simulink model "fft_biplex_real_4x_delay_bram_test"  (Simulink 7.4)
settings: Solver=VariableStepDiscrete  StartTime=0.0  StopTime=256  RelTol=1e-3
libraries: xbsIndex_r4 x596, casper_library_misc x36, casper_library_delays x8, casper_library_ffts_twiddle x1, simulink x1
(part 3 of 6)

== system fft_biplex_real_4x_delay_bram_test/fft_biplex_real_4x/biplex_core/fft_stage_3 ==
  in1 : Inport  OutDataType=sfix(16)  OutScaling=2^0
  in2 : Inport  Port=2  OutDataType=sfix(16)  OutScaling=2^0
  of_in : Inport  Port=3  OutDataType=sfix(16)  OutScaling=2^0
  sync : Inport  Port=4  OutDataType=sfix(16)  OutScaling=2^0
  shift : Inport  Port=5  OutDataType=sfix(16)  OutScaling=2^0
  Counter : xbsIndex_r4/Counter  cnt_type=Free Running  cnt_to=Inf  operation=Up  start_count=0  cnt_by_val=1  arith_type=Unsigned  n_bits=FFTSize-FFTStage+1  bin_pt=0  load_pin=off  rst=on  en=off  explicit_period=off  period=1  dbl_ovrd=off  use_behavioral_HDL=off  implementation=Fabric  use_rpm=off  block_type=counter
      settings: xl_area=[0, 0, 0, 0, 0, 0, 0]  block_version=9.1.01
  Delay : xbsIndex_r4/Delay  en=off  latency=1  dbl_ovrd=off  reg_retiming=off  block_type=delay
      settings: xl_area=[0, 0, 0, 0, 0, 0, 0]  block_version=9.1.01
  Logical1 : xbsIndex_r4/Logical  logical_function=OR  inputs=2  en=off  latency=1  precision=Full  arith_type=Unsigned  n_bits=8  bin_pt=2  align_bp=on  dbl_ovrd=off  block_type=logical
      settings: xl_area=[0, 0, 0, 0, 0, 0, 0]  block_version=9.1.01
  Mux : xbsIndex_r4/Mux  inputs=2  en=off  latency=1  precision=Full  arith_type="Signed  (2's comp)"  n_bits=8  bin_pt=2  quantization=Truncate  overflow=Wrap  dbl_ovrd=off  block_type=mux
      settings: xl_area=[0, 0, 0, 0, 0, 0, 0]  block_version=9.1.01
  Mux1 : xbsIndex_r4/Mux  inputs=2  en=off  latency=1  precision=Full  arith_type="Signed  (2's comp)"  n_bits=8  bin_pt=2  quantization=Truncate  overflow=Wrap  dbl_ovrd=off  block_type=mux
      settings: xl_area=[0, 0, 0, 0, 0, 0, 0]  block_version=9.1.01
  Slice : xbsIndex_r4/Slice  nbits=1  boolean_output=on  mode=Lower Bit Location + Width  bit1=-(FFTStage - 1)  base1=MSB of Input  bit0=FFTStage - 1  base0=LSB of Input  dbl_ovrd=off  block_type=slice
      settings: infoedit="Extracts a given range of bits from each input sample and presents it at the output.  The output type is ordinarily unsigned with binary point at zero, but can be Boolean when the slice is one bit wide.<P><P>Hardware notes: In hardware this block costs nothing."  block_version=9.1.01
  Slice1 : xbsIndex_r4/Slice  nbits=1  boolean_output=off  mode=Upper Bit Location + Width  bit1=0  base1=MSB of Input  bit0=0  base0=LSB of Input  dbl_ovrd=off  block_type=slice
      settings: infoedit="Extracts a given range of bits from each input sample and presents it at the output.  The output type is ordinarily unsigned with binary point at zero, but can be Boolean when the slice is one bit wide.<P><P>Hardware notes: In hardware this block costs nothing."  block_version=9.1.01
  butterfly_direct : Subsystem  AncestorBlock=casper_library_ffts/butterfly_direct  mask(butterfly_direct){biplex=on, FFTSize=5, Coeffs=getfield( getfield( get_param( gcb,'UserData' ), 'parameters'),'Coeffs'), StepPeriod=2, coeff_bit_width=16, input_bit_width=16, downshift=off, add_latency=1, mult_latency=3, bram_latency=1, conv_latency=2, quantization=Truncate, overflow=Saturate, arch=Virtex2Pro, opt_target=multipliers, coeffs_bram=off, use_hdl=on, use_embedded=off, hardcode_shifts=off, dsp48_adders=off}
      mask prompts: biplex "Used in biplex FFT"; FFTSize "Size of FFT: (2^? pts)"; Coeffs "Coefficients: (0 to 2^(FFTSize-1)-1)"; StepPeriod "Coefficient Step Period: (2^?)"; coeff_bit_width "Coefficient Bit Width"; input_bit_width "Input/Output Bit Width:"; add_latency "Add Latency"; mult_latency "Mult Latency"; bram_latency "BRAM Latency"; conv_latency "Convert latency"; quantization "Quantization Behavior"; overflow "Overflow Behavior"; arch "Architecture"; opt_target "Use less"; coeffs_bram "Store coefficients in BRAM"; use_hdl "Use behavioural HDL for multipliers"; use_embedded "Use embedded multipliers"; hardcode_shifts "Hardcode shift schedule"; dsp48_adders "Use DSP48s for adders"
      mask help: FFT internal block.
      mask init: same as fft_biplex_real_4x_delay_bram_test/fft_biplex_real_4x/biplex_core/fft_stage_1/butterfly_direct
      settings: AttributesFormatString=|
      | twiddle_general_3mult
      | coeffs in slices
      mask StyleString: checkbox,edit,edit,edit,edit,edit,checkbox,edit,edit,edit,edit,popup(Truncate|Round  (unbiased: +/- Inf)|Round  (unbiased: Even Values)),popup(Wrap|Saturate|Error),popup(Virtex2Pro|Virtex5),popup(logic|multipliers),checkbox,checkbox,checkbox,checkbox,checkbox
      mask CallbackString:
      | ||Coeffs = get_param(gcb, 'Coeffs');
      | if (length(eval(Coeffs)) == 1),
      |     set_param_state(gcb, 'StepPeriod', 'off');
      |     set_param_state(gcb, 'coeffs_bram', 'off');
      |     set_param_state(gcb, 'coeff_bit_width', 'off');
      | else
      |     set_param_state(gcb, 'StepPeriod', 'on');
      |     set_param_state(gcb, 'coeffs_bram', 'on');
      |     set_param_state(gcb, 'coeff_bit_width', 'on');
      | end|||||||||||fft_callback_arch(gcb);|||% make mutually exclusive with use_embedded.
      | 
      | use_hdl = get_param(gcb, 'use_hdl');
      | if strcmp(use_hdl, 'on'),
      |     set_param_state(gcb, 'use_embedded', 'off');
      | else
      |     set_param_state(gcb, 'use_embedded', 'on');
      | end|% make mutually exclusive with use_hdl.
      | 
      | use_hdl = get_param(gcb, 'use_embedded');
      | if strcmp(use_hdl, 'on'),
      |     set_param_state(gcb, 'use_hdl', 'off');
      | else
      |     set_param_state(gcb, 'use_hdl', 'on');
      | end|hardcode_shifts = get_param(gcb, 'hardcode_shifts');
      | set_param_state(gcb, 'downshift', hardcode_shifts);|fft_callback_dsp48_adders(gcb);
      mask TabNameString: Basic,Basic,Basic,Basic,Basic,Basic,Basic,Latency,Latency,Latency,Latency,Implementation,Implementation,Implementation,Implementation,Implementation,Implementation,Implementation,Implementation,Implementation
  delay_b : Subsystem  AncestorBlock=casper_library_delays/delay_slr  mask(delay_slr){DelayLen=2^(FFTSize-FFTStage)}
      mask prompts: DelayLen "Delay by:"
      mask help: A delay block that uses slices (SLR16s) for its storage.
      mask Help: eval('xlWeb(''http://casper.berkeley.edu/wiki/Delay_slr'')')
  delay_f : Subsystem  AncestorBlock=casper_library_delays/delay_slr  mask(delay_slr){DelayLen=2^(FFTSize-FFTStage)}
      mask prompts: DelayLen "Delay by:"
      mask help: A delay block that uses slices (SLR16s) for its storage.
      mask Help: eval('xlWeb(''http://casper.berkeley.edu/wiki/Delay_slr'')')
  sync_delay : casper_library_delays/sync_delay  SystemSampleTime=-1  DelayLen=2^(FFTSize - FFTStage)
  out1 : Outport  OutDataType=sfix(16)  OutScaling=2^0
  out2 : Outport  Port=2  OutDataType=sfix(16)  OutScaling=2^0
  of : Outport  Port=3  OutDataType=sfix(16)  OutScaling=2^0
  sync_out : Outport  Port=4  OutDataType=sfix(16)  OutScaling=2^0
  wires:
  shift/1 -> Slice/1
  of_in/1 -> Logical1/2
  Logical1/1 -> of/1
  Delay/1 -> sync_delay/1
  sync/1 -> Counter/1, Delay/1
  Counter/1 -> Slice1/1
  Mux/1 -> butterfly_direct/2(b)
  Mux1/1 -> delay_b/1(In1)
  delay_f/1(Out1) -> Mux1/3, Mux/2
  in1/1 -> Mux/3, Mux1/2
  Slice1/1 -> Mux/1, Mux1/1
  in2/1 -> delay_f/1(In1)
  delay_b/1(Out1) -> butterfly_direct/1(a)
  sync_delay/1 -> butterfly_direct/3(sync)
  Slice/1 -> butterfly_direct/4(shift)
  butterfly_direct/1(a+bw) -> out1/1
  butterfly_direct/2(a-bw) -> out2/1
  butterfly_direct/3(of) -> Logical1/1
  butterfly_direct/4(sync_out) -> sync_out/1

== system fft_biplex_real_4x_delay_bram_test/fft_biplex_real_4x/biplex_core/fft_stage_4 ==
  in1 : Inport  OutDataType=sfix(16)  OutScaling=2^0
  in2 : Inport  Port=2  OutDataType=sfix(16)  OutScaling=2^0
  of_in : Inport  Port=3  OutDataType=sfix(16)  OutScaling=2^0
  sync : Inport  Port=4  OutDataType=sfix(16)  OutScaling=2^0
  shift : Inport  Port=5  OutDataType=sfix(16)  OutScaling=2^0
  Counter : xbsIndex_r4/Counter  cnt_type=Free Running  cnt_to=Inf  operation=Up  start_count=0  cnt_by_val=1  arith_type=Unsigned  n_bits=FFTSize-FFTStage+1  bin_pt=0  load_pin=off  rst=on  en=off  explicit_period=off  period=1  dbl_ovrd=off  use_behavioral_HDL=off  implementation=Fabric  use_rpm=off  block_type=counter
      settings: xl_area=[0, 0, 0, 0, 0, 0, 0]  block_version=9.1.01
  Delay : xbsIndex_r4/Delay  en=off  latency=1  dbl_ovrd=off  reg_retiming=off  block_type=delay
      settings: xl_area=[0, 0, 0, 0, 0, 0, 0]  block_version=9.1.01
  Logical1 : xbsIndex_r4/Logical  logical_function=OR  inputs=2  en=off  latency=1  precision=Full  arith_type=Unsigned  n_bits=8  bin_pt=2  align_bp=on  dbl_ovrd=off  block_type=logical
      settings: xl_area=[0, 0, 0, 0, 0, 0, 0]  block_version=9.1.01
  Mux : xbsIndex_r4/Mux  inputs=2  en=off  latency=1  precision=Full  arith_type="Signed  (2's comp)"  n_bits=8  bin_pt=2  quantization=Truncate  overflow=Wrap  dbl_ovrd=off  block_type=mux
      settings: xl_area=[0, 0, 0, 0, 0, 0, 0]  block_version=9.1.01
  Mux1 : xbsIndex_r4/Mux  inputs=2  en=off  latency=1  precision=Full  arith_type="Signed  (2's comp)"  n_bits=8  bin_pt=2  quantization=Truncate  overflow=Wrap  dbl_ovrd=off  block_type=mux
      settings: xl_area=[0, 0, 0, 0, 0, 0, 0]  block_version=9.1.01
  Slice : xbsIndex_r4/Slice  nbits=1  boolean_output=on  mode=Lower Bit Location + Width  bit1=-(FFTStage - 1)  base1=MSB of Input  bit0=FFTStage - 1  base0=LSB of Input  dbl_ovrd=off  block_type=slice
      settings: infoedit="Extracts a given range of bits from each input sample and presents it at the output.  The output type is ordinarily unsigned with binary point at zero, but can be Boolean when the slice is one bit wide.<P><P>Hardware notes: In hardware this block costs nothing."  block_version=9.1.01
  Slice1 : xbsIndex_r4/Slice  nbits=1  boolean_output=off  mode=Upper Bit Location + Width  bit1=0  base1=MSB of Input  bit0=0  base0=LSB of Input  dbl_ovrd=off  block_type=slice
      settings: infoedit="Extracts a given range of bits from each input sample and presents it at the output.  The output type is ordinarily unsigned with binary point at zero, but can be Boolean when the slice is one bit wide.<P><P>Hardware notes: In hardware this block costs nothing."  block_version=9.1.01
  butterfly_direct : Subsystem  AncestorBlock=casper_library_ffts/butterfly_direct  mask(butterfly_direct){biplex=on, FFTSize=5, Coeffs=getfield( getfield( get_param( gcb,'UserData' ), 'parameters'),'Coeffs'), StepPeriod=1, coeff_bit_width=16, input_bit_width=16, downshift=off, add_latency=1, mult_latency=3, bram_latency=1, conv_latency=2, quantization=Truncate, overflow=Saturate, arch=Virtex2Pro, opt_target=multipliers, coeffs_bram=off, use_hdl=on, use_embedded=off, hardcode_shifts=off, dsp48_adders=off}
      mask prompts: biplex "Used in biplex FFT"; FFTSize "Size of FFT: (2^? pts)"; Coeffs "Coefficients: (0 to 2^(FFTSize-1)-1)"; StepPeriod "Coefficient Step Period: (2^?)"; coeff_bit_width "Coefficient Bit Width"; input_bit_width "Input/Output Bit Width:"; add_latency "Add Latency"; mult_latency "Mult Latency"; bram_latency "BRAM Latency"; conv_latency "Convert latency"; quantization "Quantization Behavior"; overflow "Overflow Behavior"; arch "Architecture"; opt_target "Use less"; coeffs_bram "Store coefficients in BRAM"; use_hdl "Use behavioural HDL for multipliers"; use_embedded "Use embedded multipliers"; hardcode_shifts "Hardcode shift schedule"; dsp48_adders "Use DSP48s for adders"
      mask help: FFT internal block.
      mask init: same as fft_biplex_real_4x_delay_bram_test/fft_biplex_real_4x/biplex_core/fft_stage_1/butterfly_direct
      settings: AttributesFormatString=|
      | twiddle_general_3mult
      | coeffs in slices
      mask StyleString: checkbox,edit,edit,edit,edit,edit,checkbox,edit,edit,edit,edit,popup(Truncate|Round  (unbiased: +/- Inf)|Round  (unbiased: Even Values)),popup(Wrap|Saturate|Error),popup(Virtex2Pro|Virtex5),popup(logic|multipliers),checkbox,checkbox,checkbox,checkbox,checkbox
      mask CallbackString:
      | ||Coeffs = get_param(gcb, 'Coeffs');
      | if (length(eval(Coeffs)) == 1),
      |     set_param_state(gcb, 'StepPeriod', 'off');
      |     set_param_state(gcb, 'coeffs_bram', 'off');
      |     set_param_state(gcb, 'coeff_bit_width', 'off');
      | else
      |     set_param_state(gcb, 'StepPeriod', 'on');
      |     set_param_state(gcb, 'coeffs_bram', 'on');
      |     set_param_state(gcb, 'coeff_bit_width', 'on');
      | end|||||||||||fft_callback_arch(gcb);|||% make mutually exclusive with use_embedded.
      | 
      | use_hdl = get_param(gcb, 'use_hdl');
      | if strcmp(use_hdl, 'on'),
      |     set_param_state(gcb, 'use_embedded', 'off');
      | else
      |     set_param_state(gcb, 'use_embedded', 'on');
      | end|% make mutually exclusive with use_hdl.
      | 
      | use_hdl = get_param(gcb, 'use_embedded');
      | if strcmp(use_hdl, 'on'),
      |     set_param_state(gcb, 'use_hdl', 'off');
      | else
      |     set_param_state(gcb, 'use_hdl', 'on');
      | end|hardcode_shifts = get_param(gcb, 'hardcode_shifts');
      | set_param_state(gcb, 'downshift', hardcode_shifts);|fft_callback_dsp48_adders(gcb);
      mask TabNameString: Basic,Basic,Basic,Basic,Basic,Basic,Basic,Latency,Latency,Latency,Latency,Implementation,Implementation,Implementation,Implementation,Implementation,Implementation,Implementation,Implementation,Implementation
  delay_b : Subsystem  AncestorBlock=casper_library_delays/delay_slr  mask(delay_slr){DelayLen=2^(FFTSize-FFTStage)}
      mask prompts: DelayLen "Delay by:"
      mask help: A delay block that uses slices (SLR16s) for its storage.
      mask Help: eval('xlWeb(''http://casper.berkeley.edu/wiki/Delay_slr'')')
  delay_f : Subsystem  AncestorBlock=casper_library_delays/delay_slr  mask(delay_slr){DelayLen=2^(FFTSize-FFTStage)}
      mask prompts: DelayLen "Delay by:"
      mask help: A delay block that uses slices (SLR16s) for its storage.
      mask Help: eval('xlWeb(''http://casper.berkeley.edu/wiki/Delay_slr'')')
  sync_delay : casper_library_delays/sync_delay  SystemSampleTime=-1  DelayLen=2^(FFTSize - FFTStage)
  out1 : Outport  OutDataType=sfix(16)  OutScaling=2^0
  out2 : Outport  Port=2  OutDataType=sfix(16)  OutScaling=2^0
  of : Outport  Port=3  OutDataType=sfix(16)  OutScaling=2^0
  sync_out : Outport  Port=4  OutDataType=sfix(16)  OutScaling=2^0
  wires:
  shift/1 -> Slice/1
  of_in/1 -> Logical1/2
  Logical1/1 -> of/1
  Delay/1 -> sync_delay/1
  sync/1 -> Counter/1, Delay/1
  Counter/1 -> Slice1/1
  Mux/1 -> butterfly_direct/2(b)
  Mux1/1 -> delay_b/1(In1)
  delay_f/1(Out1) -> Mux1/3, Mux/2
  in1/1 -> Mux/3, Mux1/2
  Slice1/1 -> Mux/1, Mux1/1
  in2/1 -> delay_f/1(In1)
  delay_b/1(Out1) -> butterfly_direct/1(a)
  sync_delay/1 -> butterfly_direct/3(sync)
  Slice/1 -> butterfly_direct/4(shift)
  butterfly_direct/1(a+bw) -> out1/1
  butterfly_direct/2(a-bw) -> out2/1
  butterfly_direct/3(of) -> Logical1/1
  butterfly_direct/4(sync_out) -> sync_out/1

== system fft_biplex_real_4x_delay_bram_test/fft_biplex_real_4x/biplex_core/fft_stage_5 ==
  in1 : Inport  OutDataType=sfix(16)  OutScaling=2^0
  in2 : Inport  Port=2  OutDataType=sfix(16)  OutScaling=2^0
  of_in : Inport  Port=3  OutDataType=sfix(16)  OutScaling=2^0
  sync : Inport  Port=4  OutDataType=sfix(16)  OutScaling=2^0
  shift : Inport  Port=5  OutDataType=sfix(16)  OutScaling=2^0
  Counter : xbsIndex_r4/Counter  cnt_type=Free Running  cnt_to=Inf  operation=Up  start_count=0  cnt_by_val=1  arith_type=Unsigned  n_bits=FFTSize-FFTStage+1  bin_pt=0  load_pin=off  rst=on  en=off  explicit_period=off  period=1  dbl_ovrd=off  use_behavioral_HDL=off  implementation=Fabric  use_rpm=off  block_type=counter
      settings: xl_area=[0, 0, 0, 0, 0, 0, 0]  block_version=9.1.01
  Delay : xbsIndex_r4/Delay  en=off  latency=1  dbl_ovrd=off  reg_retiming=off  block_type=delay
      settings: xl_area=[0, 0, 0, 0, 0, 0, 0]  block_version=9.1.01
  Logical1 : xbsIndex_r4/Logical  logical_function=OR  inputs=2  en=off  latency=1  precision=Full  arith_type=Unsigned  n_bits=8  bin_pt=2  align_bp=on  dbl_ovrd=off  block_type=logical
      settings: xl_area=[0, 0, 0, 0, 0, 0, 0]  block_version=9.1.01
  Mux : xbsIndex_r4/Mux  inputs=2  en=off  latency=1  precision=Full  arith_type="Signed  (2's comp)"  n_bits=8  bin_pt=2  quantization=Truncate  overflow=Wrap  dbl_ovrd=off  block_type=mux
      settings: xl_area=[0, 0, 0, 0, 0, 0, 0]  block_version=9.1.01
  Mux1 : xbsIndex_r4/Mux  inputs=2  en=off  latency=1  precision=Full  arith_type="Signed  (2's comp)"  n_bits=8  bin_pt=2  quantization=Truncate  overflow=Wrap  dbl_ovrd=off  block_type=mux
      settings: xl_area=[0, 0, 0, 0, 0, 0, 0]  block_version=9.1.01
  Slice : xbsIndex_r4/Slice  nbits=1  boolean_output=on  mode=Lower Bit Location + Width  bit1=-(FFTStage - 1)  base1=MSB of Input  bit0=FFTStage - 1  base0=LSB of Input  dbl_ovrd=off  block_type=slice
      settings: infoedit="Extracts a given range of bits from each input sample and presents it at the output.  The output type is ordinarily unsigned with binary point at zero, but can be Boolean when the slice is one bit wide.<P><P>Hardware notes: In hardware this block costs nothing."  block_version=9.1.01
  Slice1 : xbsIndex_r4/Slice  nbits=1  boolean_output=off  mode=Upper Bit Location + Width  bit1=0  base1=MSB of Input  bit0=0  base0=LSB of Input  dbl_ovrd=off  block_type=slice
      settings: infoedit="Extracts a given range of bits from each input sample and presents it at the output.  The output type is ordinarily unsigned with binary point at zero, but can be Boolean when the slice is one bit wide.<P><P>Hardware notes: In hardware this block costs nothing."  block_version=9.1.01
  butterfly_direct : Subsystem  AncestorBlock=casper_library_ffts/butterfly_direct  mask(butterfly_direct){biplex=on, FFTSize=5, Coeffs=getfield( getfield( get_param( gcb,'UserData' ), 'parameters'),'Coeffs'), StepPeriod=0, coeff_bit_width=16, input_bit_width=16, downshift=off, add_latency=1, mult_latency=3, bram_latency=1, conv_latency=2, quantization=Truncate, overflow=Saturate, arch=Virtex2Pro, opt_target=multipliers, coeffs_bram=off, use_hdl=off, use_embedded=on, hardcode_shifts=off, dsp48_adders=off}
      mask prompts: biplex "Used in biplex FFT"; FFTSize "Size of FFT: (2^? pts)"; Coeffs "Coefficients: (0 to 2^(FFTSize-1)-1)"; StepPeriod "Coefficient Step Period: (2^?)"; coeff_bit_width "Coefficient Bit Width"; input_bit_width "Input/Output Bit Width:"; add_latency "Add Latency"; mult_latency "Mult Latency"; bram_latency "BRAM Latency"; conv_latency "Convert latency"; quantization "Quantization Behavior"; overflow "Overflow Behavior"; arch "Architecture"; opt_target "Use less"; coeffs_bram "Store coefficients in BRAM"; use_hdl "Use behavioural HDL for multipliers"; use_embedded "Use embedded multipliers"; hardcode_shifts "Hardcode shift schedule"; dsp48_adders "Use DSP48s for adders"
      mask help: FFT internal block.
      mask init: same as fft_biplex_real_4x_delay_bram_test/fft_biplex_real_4x/biplex_core/fft_stage_1/butterfly_direct
      settings: AttributesFormatString=|
      | twiddle_general_3mult
      | coeffs in slices
      mask StyleString: checkbox,edit,edit,edit,edit,edit,checkbox,edit,edit,edit,edit,popup(Truncate|Round  (unbiased: +/- Inf)|Round  (unbiased: Even Values)),popup(Wrap|Saturate|Error),popup(Virtex2Pro|Virtex5),popup(logic|multipliers),checkbox,checkbox,checkbox,checkbox,checkbox
      mask CallbackString:
      | ||Coeffs = get_param(gcb, 'Coeffs');
      | if (length(eval(Coeffs)) == 1),
      |     set_param_state(gcb, 'StepPeriod', 'off');
      |     set_param_state(gcb, 'coeffs_bram', 'off');
      |     set_param_state(gcb, 'coeff_bit_width', 'off');
      | else
      |     set_param_state(gcb, 'StepPeriod', 'on');
      |     set_param_state(gcb, 'coeffs_bram', 'on');
      |     set_param_state(gcb, 'coeff_bit_width', 'on');
      | end|||||||||||fft_callback_arch(gcb);|||% make mutually exclusive with use_embedded.
      | 
      | use_hdl = get_param(gcb, 'use_hdl');
      | if strcmp(use_hdl, 'on'),
      |     set_param_state(gcb, 'use_embedded', 'off');
      | else
      |     set_param_state(gcb, 'use_embedded', 'on');
      | end|% make mutually exclusive with use_hdl.
      | 
      | use_hdl = get_param(gcb, 'use_embedded');
      | if strcmp(use_hdl, 'on'),
      |     set_param_state(gcb, 'use_hdl', 'off');
      | else
      |     set_param_state(gcb, 'use_hdl', 'on');
      | end|hardcode_shifts = get_param(gcb, 'hardcode_shifts');
      | set_param_state(gcb, 'downshift', hardcode_shifts);|fft_callback_dsp48_adders(gcb);
      mask TabNameString: Basic,Basic,Basic,Basic,Basic,Basic,Basic,Latency,Latency,Latency,Latency,Implementation,Implementation,Implementation,Implementation,Implementation,Implementation,Implementation,Implementation,Implementation
  delay_b : Subsystem  AncestorBlock=casper_library_delays/delay_slr  mask(delay_slr){DelayLen=2^(FFTSize-FFTStage)}
      mask prompts: DelayLen "Delay by:"
      mask help: A delay block that uses slices (SLR16s) for its storage.
      mask Help: eval('xlWeb(''http://casper.berkeley.edu/wiki/Delay_slr'')')
  delay_f : Subsystem  AncestorBlock=casper_library_delays/delay_slr  mask(delay_slr){DelayLen=2^(FFTSize-FFTStage)}
      mask prompts: DelayLen "Delay by:"
      mask help: A delay block that uses slices (SLR16s) for its storage.
      mask Help: eval('xlWeb(''http://casper.berkeley.edu/wiki/Delay_slr'')')
  sync_delay : casper_library_delays/sync_delay  SystemSampleTime=-1  DelayLen=2^(FFTSize - FFTStage)
  out1 : Outport  OutDataType=sfix(16)  OutScaling=2^0
  out2 : Outport  Port=2  OutDataType=sfix(16)  OutScaling=2^0
  of : Outport  Port=3  OutDataType=sfix(16)  OutScaling=2^0
  sync_out : Outport  Port=4  OutDataType=sfix(16)  OutScaling=2^0
  wires:
  shift/1 -> Slice/1
  of_in/1 -> Logical1/2
  Logical1/1 -> of/1
  Delay/1 -> sync_delay/1
  sync/1 -> Counter/1, Delay/1
  Counter/1 -> Slice1/1
  Mux/1 -> butterfly_direct/2(b)
  Mux1/1 -> delay_b/1(In1)
  delay_f/1(Out1) -> Mux1/3, Mux/2
  in1/1 -> Mux/3, Mux1/2
  Slice1/1 -> Mux/1, Mux1/1
  in2/1 -> delay_f/1(In1)
  delay_b/1(Out1) -> butterfly_direct/1(a)
  sync_delay/1 -> butterfly_direct/3(sync)
  Slice/1 -> butterfly_direct/4(shift)
  butterfly_direct/1(a+bw) -> out1/1
  butterfly_direct/2(a-bw) -> out2/1
  butterfly_direct/3(of) -> Logical1/1
  butterfly_direct/4(sync_out) -> sync_out/1

== system fft_biplex_real_4x_delay_bram_test/fft_biplex_real_4x/bi_real_unscr_4x/hilbert0/c_to_ri ==
  c : Inport  OutDataType=sfix(16)  OutScaling=2^0
  force_im : xbsIndex_r4/Reinterpret  force_arith_type=on  arith_type="Signed  (2's comp)"  force_bin_pt=on  bin_pt=bin_pt  block_type=reinterpret
      settings: infoedit="Changes signal type without altering the binary representation.   You can changed the signal between signed and unsigned, and relocate the binary point.<P><P>Hardware notes: In hardware this block costs nothing.<P><P>Example:  Suppose the input is 6 bits wide, signed, with 2 fractional bits, and the output is forced to unsigned with 0 fractional bits.  Then an input of -2.0 (1110.00 in binary 2's complement) becomes an output of 56 (111000 in binary)."  block_version=9.1.01
  force_re : xbsIndex_r4/Reinterpret  force_arith_type=on  arith_type="Signed  (2's comp)"  force_bin_pt=on  bin_pt=bin_pt  block_type=reinterpret
      settings: infoedit="Changes signal type without altering the binary representation.   You can changed the signal between signed and unsigned, and relocate the binary point.<P><P>Hardware notes: In hardware this block costs nothing.<P><P>Example:  Suppose the input is 6 bits wide, signed, with 2 fractional bits, and the output is forced to unsigned with 0 fractional bits.  Then an input of -2.0 (1110.00 in binary 2's complement) becomes an output of 56 (111000 in binary)."  block_version=9.1.01
  slice_im : xbsIndex_r4/Slice  nbits=n_bits  boolean_output=off  mode=Lower Bit Location + Width  bit1=0  base1=MSB of Input  bit0=0  base0=LSB of Input  dbl_ovrd=off  block_type=slice
      settings: infoedit="Extracts a given range of bits from each input sample and presents it at the output.  The output type is ordinarily unsigned with binary point at zero, but can be Boolean when the slice is one bit wide.<P><P>Hardware notes: In hardware this block costs nothing."  block_version=9.1.01
  slice_re : xbsIndex_r4/Slice  nbits=n_bits  boolean_output=off  mode=Upper Bit Location + Width  bit1=0  base1=MSB of Input  bit0=0  base0=LSB of Input  dbl_ovrd=off  block_type=slice
      settings: infoedit="Extracts a given range of bits from each input sample and presents it at the output.  The output type is ordinarily unsigned with binary point at zero, but can be Boolean when the slice is one bit wide.<P><P>Hardware notes: In hardware this block costs nothing."  block_version=9.1.01
  re : Outport  OutDataType=sfix(16)  OutScaling=2^0
  im : Outport  Port=2  OutDataType=sfix(16)  OutScaling=2^0
  wires:
  slice_re/1 -> force_re/1
  slice_im/1 -> force_im/1
  force_re/1 -> re/1
  force_im/1 -> im/1
  c/1 -> slice_re/1, slice_im/1

== system fft_biplex_real_4x_delay_bram_test/fft_biplex_real_4x/bi_real_unscr_4x/hilbert0/c_to_ri1 ==
  c : Inport  OutDataType=sfix(16)  OutScaling=2^0
  force_im : xbsIndex_r4/Reinterpret  force_arith_type=on  arith_type="Signed  (2's comp)"  force_bin_pt=on  bin_pt=bin_pt  block_type=reinterpret
      settings: infoedit="Changes signal type without altering the binary representation.   You can changed the signal between signed and unsigned, and relocate the binary point.<P><P>Hardware notes: In hardware this block costs nothing.<P><P>Example:  Suppose the input is 6 bits wide, signed, with 2 fractional bits, and the output is forced to unsigned with 0 fractional bits.  Then an input of -2.0 (1110.00 in binary 2's complement) becomes an output of 56 (111000 in binary)."  block_version=9.1.01
  force_re : xbsIndex_r4/Reinterpret  force_arith_type=on  arith_type="Signed  (2's comp)"  force_bin_pt=on  bin_pt=bin_pt  block_type=reinterpret
      settings: infoedit="Changes signal type without altering the binary representation.   You can changed the signal between signed and unsigned, and relocate the binary point.<P><P>Hardware notes: In hardware this block costs nothing.<P><P>Example:  Suppose the input is 6 bits wide, signed, with 2 fractional bits, and the output is forced to unsigned with 0 fractional bits.  Then an input of -2.0 (1110.00 in binary 2's complement) becomes an output of 56 (111000 in binary)."  block_version=9.1.01
  slice_im : xbsIndex_r4/Slice  nbits=n_bits  boolean_output=off  mode=Lower Bit Location + Width  bit1=0  base1=MSB of Input  bit0=0  base0=LSB of Input  dbl_ovrd=off  block_type=slice
      settings: infoedit="Extracts a given range of bits from each input sample and presents it at the output.  The output type is ordinarily unsigned with binary point at zero, but can be Boolean when the slice is one bit wide.<P><P>Hardware notes: In hardware this block costs nothing."  block_version=9.1.01
  slice_re : xbsIndex_r4/Slice  nbits=n_bits  boolean_output=off  mode=Upper Bit Location + Width  bit1=0  base1=MSB of Input  bit0=0  base0=LSB of Input  dbl_ovrd=off  block_type=slice
      settings: infoedit="Extracts a given range of bits from each input sample and presents it at the output.  The output type is ordinarily unsigned with binary point at zero, but can be Boolean when the slice is one bit wide.<P><P>Hardware notes: In hardware this block costs nothing."  block_version=9.1.01
  re : Outport  OutDataType=sfix(16)  OutScaling=2^0
  im : Outport  Port=2  OutDataType=sfix(16)  OutScaling=2^0
  wires:
  slice_re/1 -> force_re/1
  slice_im/1 -> force_im/1
  force_re/1 -> re/1
  force_im/1 -> im/1
  c/1 -> slice_re/1, slice_im/1

== system fft_biplex_real_4x_delay_bram_test/fft_biplex_real_4x/bi_real_unscr_4x/hilbert0/ri_to_c ==
  re : Inport  OutDataType=sfix(16)  OutScaling=2^0
  im : Inport  Port=2  OutDataType=sfix(16)  OutScaling=2^0
  concat : xbsIndex_r4/Concat  num_inputs=2  dbl_ovrd=off  block_type=concat
      settings: block_version=9.1.01
  force_im : xbsIndex_r4/Reinterpret  force_arith_type=on  arith_type=Unsigned  force_bin_pt=on  bin_pt=0  block_type=reinterpret
      settings: infoedit="Changes signal type without altering the binary representation.   You can changed the signal between signed and unsigned, and relocate the binary point.<P><P>Hardware notes: In hardware this block costs nothing.<P><P>Example:  Suppose the input is 6 bits wide, signed, with 2 fractional bits, and the output is forced to unsigned with 0 fractional bits.  Then an input of -2.0 (1110.00 in binary 2's complement) becomes an output of 56 (111000 in binary)."  block_version=9.1.01
  force_re : xbsIndex_r4/Reinterpret  force_arith_type=on  arith_type=Unsigned  force_bin_pt=on  bin_pt=0  block_type=reinterpret
      settings: infoedit="Changes signal type without altering the binary representation.   You can changed the signal between signed and unsigned, and relocate the binary point.<P><P>Hardware notes: In hardware this block costs nothing.<P><P>Example:  Suppose the input is 6 bits wide, signed, with 2 fractional bits, and the output is forced to unsigned with 0 fractional bits.  Then an input of -2.0 (1110.00 in binary 2's complement) becomes an output of 56 (111000 in binary)."  block_version=9.1.01
  c : Outport  OutDataType=sfix(16)  OutScaling=2^0
  wires:
  force_re/1 -> concat/1
  force_im/1 -> concat/2
  re/1 -> force_re/1
  concat/1 -> c/1
  im/1 -> force_im/1

== system fft_biplex_real_4x_delay_bram_test/fft_biplex_real_4x/bi_real_unscr_4x/hilbert0/ri_to_c1 ==
  re : Inport  OutDataType=sfix(16)  OutScaling=2^0
  im : Inport  Port=2  OutDataType=sfix(16)  OutScaling=2^0
  concat : xbsIndex_r4/Concat  num_inputs=2  dbl_ovrd=off  block_type=concat
      settings: block_version=9.1.01
  force_im : xbsIndex_r4/Reinterpret  force_arith_type=on  arith_type=Unsigned  force_bin_pt=on  bin_pt=0  block_type=reinterpret
      settings: infoedit="Changes signal type without altering the binary representation.   You can changed the signal between signed and unsigned, and relocate the binary point.<P><P>Hardware notes: In hardware this block costs nothing.<P><P>Example:  Suppose the input is 6 bits wide, signed, with 2 fractional bits, and the output is forced to unsigned with 0 fractional bits.  Then an input of -2.0 (1110.00 in binary 2's complement) becomes an output of 56 (111000 in binary)."  block_version=9.1.01
  force_re : xbsIndex_r4/Reinterpret  force_arith_type=on  arith_type=Unsigned  force_bin_pt=on  bin_pt=0  block_type=reinterpret
      settings: infoedit="Changes signal type without altering the binary representation.   You can changed the signal between signed and unsigned, and relocate the binary point.<P><P>Hardware notes: In hardware this block costs nothing.<P><P>Example:  Suppose the input is 6 bits wide, signed, with 2 fractional bits, and the output is forced to unsigned with 0 fractional bits.  Then an input of -2.0 (1110.00 in binary 2's complement) becomes an output of 56 (111000 in binary)."  block_version=9.1.01
  c : Outport  OutDataType=sfix(16)  OutScaling=2^0
  wires:
  force_re/1 -> concat/1
  force_im/1 -> concat/2
  re/1 -> force_re/1
  concat/1 -> c/1
  im/1 -> force_im/1

== system fft_biplex_real_4x_delay_bram_test/fft_biplex_real_4x/bi_real_unscr_4x/hilbert1/c_to_ri ==
  c : Inport  OutDataType=sfix(16)  OutScaling=2^0
  force_im : xbsIndex_r4/Reinterpret  force_arith_type=on  arith_type="Signed  (2's comp)"  force_bin_pt=on  bin_pt=bin_pt  block_type=reinterpret
      settings: infoedit="Changes signal type without altering the binary representation.   You can changed the signal between signed and unsigned, and relocate the binary point.<P><P>Hardware notes: In hardware this block costs nothing.<P><P>Example:  Suppose the input is 6 bits wide, signed, with 2 fractional bits, and the output is forced to unsigned with 0 fractional bits.  Then an input of -2.0 (1110.00 in binary 2's complement) becomes an output of 56 (111000 in binary)."  block_version=9.1.01
  force_re : xbsIndex_r4/Reinterpret  force_arith_type=on  arith_type="Signed  (2's comp)"  force_bin_pt=on  bin_pt=bin_pt  block_type=reinterpret
      settings: infoedit="Changes signal type without altering the binary representation.   You can changed the signal between signed and unsigned, and relocate the binary point.<P><P>Hardware notes: In hardware this block costs nothing.<P><P>Example:  Suppose the input is 6 bits wide, signed, with 2 fractional bits, and the output is forced to unsigned with 0 fractional bits.  Then an input of -2.0 (1110.00 in binary 2's complement) becomes an output of 56 (111000 in binary)."  block_version=9.1.01
  slice_im : xbsIndex_r4/Slice  nbits=n_bits  boolean_output=off  mode=Lower Bit Location + Width  bit1=0  base1=MSB of Input  bit0=0  base0=LSB of Input  dbl_ovrd=off  block_type=slice
      settings: infoedit="Extracts a given range of bits from each input sample and presents it at the output.  The output type is ordinarily unsigned with binary point at zero, but can be Boolean when the slice is one bit wide.<P><P>Hardware notes: In hardware this block costs nothing."  block_version=9.1.01
  slice_re : xbsIndex_r4/Slice  nbits=n_bits  boolean_output=off  mode=Upper Bit Location + Width  bit1=0  base1=MSB of Input  bit0=0  base0=LSB of Input  dbl_ovrd=off  block_type=slice
      settings: infoedit="Extracts a given range of bits from each input sample and presents it at the output.  The output type is ordinarily unsigned with binary point at zero, but can be Boolean when the slice is one bit wide.<P><P>Hardware notes: In hardware this block costs nothing."  block_version=9.1.01
  re : Outport  OutDataType=sfix(16)  OutScaling=2^0
  im : Outport  Port=2  OutDataType=sfix(16)  OutScaling=2^0
  wires:
  slice_re/1 -> force_re/1
  slice_im/1 -> force_im/1
  force_re/1 -> re/1
  force_im/1 -> im/1
  c/1 -> slice_re/1, slice_im/1

== system fft_biplex_real_4x_delay_bram_test/fft_biplex_real_4x/bi_real_unscr_4x/hilbert1/c_to_ri1 ==
  c : Inport  OutDataType=sfix(16)  OutScaling=2^0
  force_im : xbsIndex_r4/Reinterpret  force_arith_type=on  arith_type="Signed  (2's comp)"  force_bin_pt=on  bin_pt=bin_pt  block_type=reinterpret
      settings: infoedit="Changes signal type without altering the binary representation.   You can changed the signal between signed and unsigned, and relocate the binary point.<P><P>Hardware notes: In hardware this block costs nothing.<P><P>Example:  Suppose the input is 6 bits wide, signed, with 2 fractional bits, and the output is forced to unsigned with 0 fractional bits.  Then an input of -2.0 (1110.00 in binary 2's complement) becomes an output of 56 (111000 in binary)."  block_version=9.1.01
  force_re : xbsIndex_r4/Reinterpret  force_arith_type=on  arith_type="Signed  (2's comp)"  force_bin_pt=on  bin_pt=bin_pt  block_type=reinterpret
      settings: infoedit="Changes signal type without altering the binary representation.   You can changed the signal between signed and unsigned, and relocate the binary point.<P><P>Hardware notes: In hardware this block costs nothing.<P><P>Example:  Suppose the input is 6 bits wide, signed, with 2 fractional bits, and the output is forced to unsigned with 0 fractional bits.  Then an input of -2.0 (1110.00 in binary 2's complement) becomes an output of 56 (111000 in binary)."  block_version=9.1.01
  slice_im : xbsIndex_r4/Slice  nbits=n_bits  boolean_output=off  mode=Lower Bit Location + Width  bit1=0  base1=MSB of Input  bit0=0  base0=LSB of Input  dbl_ovrd=off  block_type=slice
      settings: infoedit="Extracts a given range of bits from each input sample and presents it at the output.  The output type is ordinarily unsigned with binary point at zero, but can be Boolean when the slice is one bit wide.<P><P>Hardware notes: In hardware this block costs nothing."  block_version=9.1.01
  slice_re : xbsIndex_r4/Slice  nbits=n_bits  boolean_output=off  mode=Upper Bit Location + Width  bit1=0  base1=MSB of Input  bit0=0  base0=LSB of Input  dbl_ovrd=off  block_type=slice
      settings: infoedit="Extracts a given range of bits from each input sample and presents it at the output.  The output type is ordinarily unsigned with binary point at zero, but can be Boolean when the slice is one bit wide.<P><P>Hardware notes: In hardware this block costs nothing."  block_version=9.1.01
  re : Outport  OutDataType=sfix(16)  OutScaling=2^0
  im : Outport  Port=2  OutDataType=sfix(16)  OutScaling=2^0
  wires:
  slice_re/1 -> force_re/1
  slice_im/1 -> force_im/1
  force_re/1 -> re/1
  force_im/1 -> im/1
  c/1 -> slice_re/1, slice_im/1

== system fft_biplex_real_4x_delay_bram_test/fft_biplex_real_4x/bi_real_unscr_4x/hilbert1/ri_to_c ==
  re : Inport  OutDataType=sfix(16)  OutScaling=2^0
  im : Inport  Port=2  OutDataType=sfix(16)  OutScaling=2^0
  concat : xbsIndex_r4/Concat  num_inputs=2  dbl_ovrd=off  block_type=concat
      settings: block_version=9.1.01
  force_im : xbsIndex_r4/Reinterpret  force_arith_type=on  arith_type=Unsigned  force_bin_pt=on  bin_pt=0  block_type=reinterpret
      settings: infoedit="Changes signal type without altering the binary representation.   You can changed the signal between signed and unsigned, and relocate the binary point.<P><P>Hardware notes: In hardware this block costs nothing.<P><P>Example:  Suppose the input is 6 bits wide, signed, with 2 fractional bits, and the output is forced to unsigned with 0 fractional bits.  Then an input of -2.0 (1110.00 in binary 2's complement) becomes an output of 56 (111000 in binary)."  block_version=9.1.01
  force_re : xbsIndex_r4/Reinterpret  force_arith_type=on  arith_type=Unsigned  force_bin_pt=on  bin_pt=0  block_type=reinterpret
      settings: infoedit="Changes signal type without altering the binary representation.   You can changed the signal between signed and unsigned, and relocate the binary point.<P><P>Hardware notes: In hardware this block costs nothing.<P><P>Example:  Suppose the input is 6 bits wide, signed, with 2 fractional bits, and the output is forced to unsigned with 0 fractional bits.  Then an input of -2.0 (1110.00 in binary 2's complement) becomes an output of 56 (111000 in binary)."  block_version=9.1.01
  c : Outport  OutDataType=sfix(16)  OutScaling=2^0
  wires:
  force_re/1 -> concat/1
  force_im/1 -> concat/2
  re/1 -> force_re/1
  concat/1 -> c/1
  im/1 -> force_im/1

== system fft_biplex_real_4x_delay_bram_test/fft_biplex_real_4x/bi_real_unscr_4x/hilbert1/ri_to_c1 ==
  re : Inport  OutDataType=sfix(16)  OutScaling=2^0
  im : Inport  Port=2  OutDataType=sfix(16)  OutScaling=2^0
  concat : xbsIndex_r4/Concat  num_inputs=2  dbl_ovrd=off  block_type=concat
      settings: block_version=9.1.01
  force_im : xbsIndex_r4/Reinterpret  force_arith_type=on  arith_type=Unsigned  force_bin_pt=on  bin_pt=0  block_type=reinterpret
      settings: infoedit="Changes signal type without altering the binary representation.   You can changed the signal between signed and unsigned, and relocate the binary point.<P><P>Hardware notes: In hardware this block costs nothing.<P><P>Example:  Suppose the input is 6 bits wide, signed, with 2 fractional bits, and the output is forced to unsigned with 0 fractional bits.  Then an input of -2.0 (1110.00 in binary 2's complement) becomes an output of 56 (111000 in binary)."  block_version=9.1.01
  force_re : xbsIndex_r4/Reinterpret  force_arith_type=on  arith_type=Unsigned  force_bin_pt=on  bin_pt=0  block_type=reinterpret
      settings: infoedit="Changes signal type without altering the binary representation.   You can changed the signal between signed and unsigned, and relocate the binary point.<P><P>Hardware notes: In hardware this block costs nothing.<P><P>Example:  Suppose the input is 6 bits wide, signed, with 2 fractional bits, and the output is forced to unsigned with 0 fractional bits.  Then an input of -2.0 (1110.00 in binary 2's complement) becomes an output of 56 (111000 in binary)."  block_version=9.1.01
  c : Outport  OutDataType=sfix(16)  OutScaling=2^0
  wires:
  force_re/1 -> concat/1
  force_im/1 -> concat/2
  re/1 -> force_re/1
  concat/1 -> c/1
  im/1 -> force_im/1

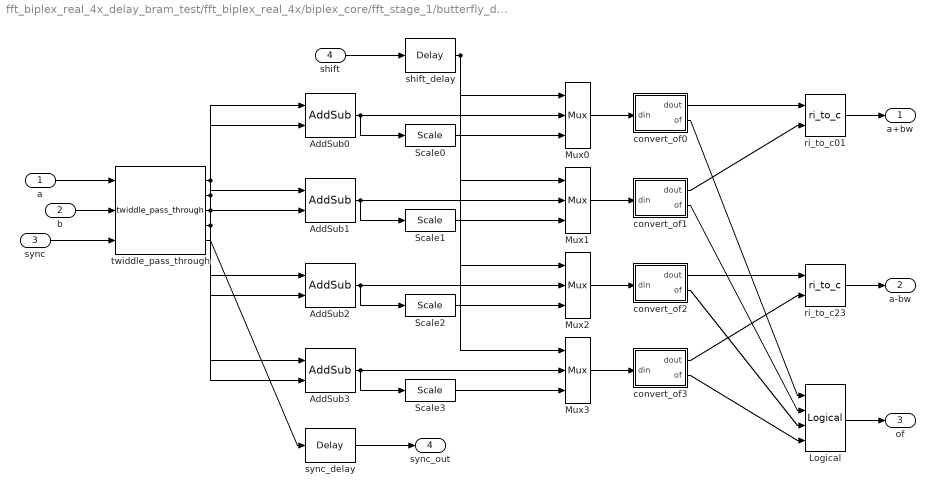
== system fft_biplex_real_4x_delay_bram_test/fft_biplex_real_4x/biplex_core/fft_stage_1/butterfly_direct ==
  a : Inport  OutDataType=sfix(16)  OutScaling=2^0
  b : Inport  Port=2  OutDataType=sfix(16)  OutScaling=2^0
  sync : Inport  Port=3  OutDataType=sfix(16)  OutScaling=2^0
  shift : Inport  Port=4  OutDataType=sfix(16)  OutScaling=2^0
  AddSub0 : xbsIndex_r4/AddSub  mode=Addition  use_carryin=off  use_carryout=off  en=off  latency=1  precision=Full  arith_type=Unsigned  n_bits=16  bin_pt=14  quantization=Truncate  overflow=Wrap  dbl_ovrd=off  use_behavioral_HDL=on  hw_selection=Fabric  pipelined=off  block_type=addsub
  AddSub1 : xbsIndex_r4/AddSub  mode=Addition  use_carryin=off  use_carryout=off  en=off  latency=1  precision=Full  arith_type=Unsigned  n_bits=16  bin_pt=14  quantization=Truncate  overflow=Wrap  dbl_ovrd=off  use_behavioral_HDL=on  hw_selection=Fabric  pipelined=off  block_type=addsub
  AddSub2 : xbsIndex_r4/AddSub  mode=Subtraction  use_carryin=off  use_carryout=off  en=off  latency=1  precision=Full  arith_type=Unsigned  n_bits=16  bin_pt=14  quantization=Truncate  overflow=Wrap  dbl_ovrd=off  use_behavioral_HDL=on  hw_selection=Fabric  pipelined=off  block_type=addsub
  AddSub3 : xbsIndex_r4/AddSub  mode=Subtraction  use_carryin=off  use_carryout=off  en=off  latency=1  precision=Full  arith_type=Unsigned  n_bits=16  bin_pt=14  quantization=Truncate  overflow=Wrap  dbl_ovrd=off  use_behavioral_HDL=on  hw_selection=Fabric  pipelined=off  block_type=addsub
  Logical : xbsIndex_r4/Logical  logical_function=OR  inputs=4  en=off  latency=0  precision=Full  arith_type=Unsigned  n_bits=16  bin_pt=0  align_bp=on  dbl_ovrd=off  block_type=logical
      settings: block_version=11.4
  Mux{0..3} (4 alike) : xbsIndex_r4/Mux  inputs=2  en=off  latency=1  precision=Full  arith_type=Unsigned  n_bits=16  bin_pt=14  quantization=Truncate  overflow=Wrap  dbl_ovrd=off  block_type=mux
      settings: block_version=11.4
  Scale{0..3} (4 alike) : xbsIndex_r4/Scale  scale_factor=-1  dbl_ovrd=off  block_type=scale
  convert_of0 : Subsystem  AncestorBlock=casper_library_misc/convert_of  mask(convert_of){bit_width_i=18, binary_point_i=16, bit_width_o=16, binary_point_o=15, latency=2, overflow=Saturate, quantization=Truncate}
      mask prompts: bit_width_i "Bit Width In"; binary_point_i "Binary Point In"; bit_width_o "Bit Width Out"; binary_point_o "Binary Point Out"; overflow "Overflow Behaviour"; quantization "Quantization Behaviour"
      mask help:
      | Converts from one 2's complement bit-width
      | and/or binary point position to another.
      | Includes underflow/overflow indicator.
      mask init:
      | convert_of_init(gcb, ...
      |     'bit_width_i', bit_width_i, ...
      |     'binary_point_i', binary_point_i, ...
      |     'bit_width_o', bit_width_o, ...
      |     'binary_point_o', binary_point_o, ...
      |     'latency', latency, ...
      |     'overflow', overflow, ...
      |     'quantization', quantization);
      settings: AttributesFormatString=[18,16]->[16,15]
      mask StyleString: edit,edit,edit,edit,edit,popup(Wrap|Saturate|Error),popup(Truncate|Round  (unbiased: +/- Inf)|Round  (unbiased: even values))
  convert_of1 : Subsystem  AncestorBlock=casper_library_misc/convert_of  mask(convert_of){bit_width_i=18, binary_point_i=16, bit_width_o=16, binary_point_o=15, latency=2, overflow=Saturate, quantization=Truncate}
      mask prompts: bit_width_i "Bit Width In"; binary_point_i "Binary Point In"; bit_width_o "Bit Width Out"; binary_point_o "Binary Point Out"; overflow "Overflow Behaviour"; quantization "Quantization Behaviour"
      mask help:
      | Converts from one 2's complement bit-width
      | and/or binary point position to another.
      | Includes underflow/overflow indicator.
      mask init: same as fft_biplex_real_4x_delay_bram_test/fft_biplex_real_4x/biplex_core/fft_stage_1/butterfly_direct/convert_of0
      settings: AttributesFormatString=[18,16]->[16,15]
      mask StyleString: edit,edit,edit,edit,edit,popup(Wrap|Saturate|Error),popup(Truncate|Round  (unbiased: +/- Inf)|Round  (unbiased: even values))
  convert_of2 : Subsystem  AncestorBlock=casper_library_misc/convert_of  mask(convert_of){bit_width_i=18, binary_point_i=16, bit_width_o=16, binary_point_o=15, latency=2, overflow=Saturate, quantization=Truncate}
      mask prompts: bit_width_i "Bit Width In"; binary_point_i "Binary Point In"; bit_width_o "Bit Width Out"; binary_point_o "Binary Point Out"; overflow "Overflow Behaviour"; quantization "Quantization Behaviour"
      mask help:
      | Converts from one 2's complement bit-width
      | and/or binary point position to another.
      | Includes underflow/overflow indicator.
      mask init: same as fft_biplex_real_4x_delay_bram_test/fft_biplex_real_4x/biplex_core/fft_stage_1/butterfly_direct/convert_of0
      settings: AttributesFormatString=[18,16]->[16,15]
      mask StyleString: edit,edit,edit,edit,edit,popup(Wrap|Saturate|Error),popup(Truncate|Round  (unbiased: +/- Inf)|Round  (unbiased: even values))
  convert_of3 : Subsystem  AncestorBlock=casper_library_misc/convert_of  mask(convert_of){bit_width_i=18, binary_point_i=16, bit_width_o=16, binary_point_o=15, latency=2, overflow=Saturate, quantization=Truncate}
      mask prompts: bit_width_i "Bit Width In"; binary_point_i "Binary Point In"; bit_width_o "Bit Width Out"; binary_point_o "Binary Point Out"; overflow "Overflow Behaviour"; quantization "Quantization Behaviour"
      mask help:
      | Converts from one 2's complement bit-width
      | and/or binary point position to another.
      | Includes underflow/overflow indicator.
      mask init: same as fft_biplex_real_4x_delay_bram_test/fft_biplex_real_4x/biplex_core/fft_stage_1/butterfly_direct/convert_of0
      settings: AttributesFormatString=[18,16]->[16,15]
      mask StyleString: edit,edit,edit,edit,edit,popup(Wrap|Saturate|Error),popup(Truncate|Round  (unbiased: +/- Inf)|Round  (unbiased: even values))
  ri_to_c01 : casper_library_misc/ri_to_c  SystemSampleTime=-1
  ri_to_c23 : casper_library_misc/ri_to_c  SystemSampleTime=-1
  shift_delay : xbsIndex_r4/Delay  en=off  latency=1  dbl_ovrd=off  reg_retiming=off  block_type=delay
      settings: block_version=11.4
  sync_delay : xbsIndex_r4/Delay  en=off  latency=4  dbl_ovrd=off  reg_retiming=on  block_type=delay
      settings: block_version=11.4
  twiddle_pass_through : casper_library_ffts_twiddle/twiddle_pass_through  SystemSampleTime=-1  FFTSize=5  input_bit_width=16  add_latency=1  mult_latency=3  bram_latency=1  conv_latency=2  opt_target=multipliers
  a+bw : Outport  OutDataType=sfix(16)  OutScaling=2^0
  a-bw : Outport  Port=2  OutDataType=sfix(16)  OutScaling=2^0
  of : Outport  Port=3  OutDataType=sfix(16)  OutScaling=2^0
  sync_out : Outport  Port=4
  wires:
  a/1 -> twiddle_pass_through/1
  b/1 -> twiddle_pass_through/2
  sync/1 -> twiddle_pass_through/3
  twiddle_pass_through/1 -> AddSub0/1, AddSub2/1
  twiddle_pass_through/2 -> AddSub1/1, AddSub3/1
  twiddle_pass_through/3 -> AddSub0/2, AddSub2/2
  twiddle_pass_through/4 -> AddSub1/2, AddSub3/2
  twiddle_pass_through/5 -> sync_delay/1
  shift/1 -> shift_delay/1
  shift_delay/1 -> Mux0/1, Mux1/1, Mux2/1, Mux3/1
  AddSub0/1 -> Mux0/2, Scale0/1
  AddSub1/1 -> Mux1/2, Scale1/1
  AddSub2/1 -> Mux2/2, Scale2/1
  AddSub3/1 -> Mux3/2, Scale3/1
  Scale0/1 -> Mux0/3
  Scale1/1 -> Mux1/3
  Scale2/1 -> Mux2/3
  Scale3/1 -> Mux3/3
  Mux0/1 -> convert_of0/1(din)
  Mux1/1 -> convert_of1/1(din)
  Mux2/1 -> convert_of2/1(din)
  Mux3/1 -> convert_of3/1(din)
  convert_of0/1(dout) -> ri_to_c01/1
  convert_of1/1(dout) -> ri_to_c01/2
  convert_of2/1(dout) -> ri_to_c23/1
  convert_of3/1(dout) -> ri_to_c23/2
  convert_of0/2(of) -> Logical/1
  convert_of1/2(of) -> Logical/2
  convert_of2/2(of) -> Logical/3
  convert_of3/2(of) -> Logical/4
  ri_to_c01/1 -> a+bw/1
  ri_to_c23/1 -> a-bw/1
  Logical/1 -> of/1
  sync_delay/1 -> sync_out/1

== system fft_biplex_real_4x_delay_bram_test/fft_biplex_real_4x/biplex_core/fft_stage_1/delay_b ==
  In1 : Inport  OutDataType=sfix(16)  OutScaling=2^0
  delay_slr : xbsIndex_r4/Delay  en=off  latency=DelayLen  dbl_ovrd=off  reg_retiming=off  block_type=delay
      settings: xl_area=[0, 0, 0, 0, 0, 0, 0]  block_version=9.1.01
  Out1 : Outport  OutDataType=sfix(16)  OutScaling=2^0
  wires:
  delay_slr/1 -> Out1/1
  In1/1 -> delay_slr/1

== system fft_biplex_real_4x_delay_bram_test/fft_biplex_real_4x/biplex_core/fft_stage_1/delay_f ==
  In1 : Inport  OutDataType=sfix(16)  OutScaling=2^0
  delay_slr : xbsIndex_r4/Delay  en=off  latency=DelayLen  dbl_ovrd=off  reg_retiming=off  block_type=delay
      settings: xl_area=[0, 0, 0, 0, 0, 0, 0]  block_version=9.1.01
  Out1 : Outport  OutDataType=sfix(16)  OutScaling=2^0
  wires:
  delay_slr/1 -> Out1/1
  In1/1 -> delay_slr/1
